simulink model "amrNavigation"  (R2025b)
settings: Solver=FixedStepDiscrete  StartTime=0.0  StopTime=119.95  FixedStep=0.050000000000000003  RelTol=1e-3
InitFcn:
  | amrModelInit
StopFcn:
  | amrModelStop
model workspace (MAT data in the model file):
  amrBuiltConstants.robot.radius = 0.22
  amrBuiltConstants.robot.wheelRadius = 0.05
  amrBuiltConstants.robot.wheelBase = 0.32
  amrBuiltConstants.robot.vMax = 0.65
  amrBuiltConstants.robot.vMin = -0.2
  amrBuiltConstants.robot.wMax = 1.4
  amrBuiltConstants.robot.aMax = 0.6
  amrBuiltConstants.robot.alphaMax = 2
  amrBuiltConstants.robot.motorTau = 0.06
  amrBuiltConstants.robot.wheelSpeedMax = 25
  amrBuiltConstants.robot.idealWheels = 0
  amrBuiltConstants.robot.integrator = 'euler'
  amrBuiltConstants.wheelPID.Kp = 0.5
  amrBuiltConstants.wheelPID.Ki = 3
  amrBuiltConstants.wheelPID.Kd = 0
  amrBuiltConstants.wheelPID.iMax = 10
  amrBuiltConstants.dt = 0.05
undefined symbols (not defined in the file or in its folder): amrStartPose
libraries: simulink x1
settings Model: Creator=kichuiyer  LastModifiedBy=kichuiyer
settings DataIOCC: SaveOutput=off  SignalLogging=off  SaveTime=off

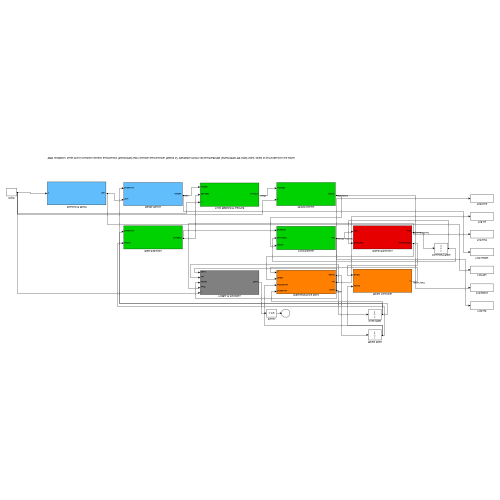
[thumbnail: Simulink's stored preview of the top-level diagram]
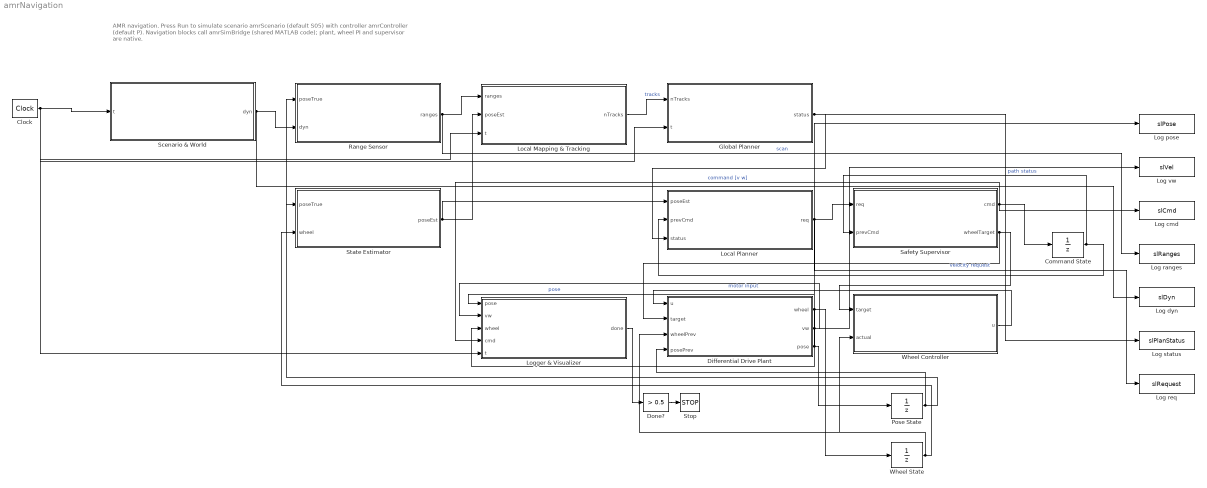
== system amrNavigation ==
  note: AMR navigation. Press Run to simulate scenario amrScenario (default S05) with controller amrController (default P). Navigation blocks call amrSimBridge (shared MATLAB code); plant, wheel PI and supervisor are native.
  Clock : DigitalClock  SampleTime=0.050000000000000003
  Command State : UnitDelay  InitialCondition=[0 0]  SampleTime=0.050000000000000003  HasFrameUpgradeWarning=on
  Differential Drive Plant : Subsystem
  Done? : simulink/Logic and Bit Operations/Compare To Constant  relop=>  const=0.5  OutDataTypeStr=boolean
  Global Planner : Subsystem
  Local Mapping & Tracking : Subsystem
  Local Planner : Subsystem
  Log cmd : ToWorkspace  VariableName=slCmd  SampleTime=-1
  Log dyn : ToWorkspace  VariableName=slDyn  SampleTime=-1
  Log pose : ToWorkspace  VariableName=slPose  SampleTime=-1
  Log ranges : ToWorkspace  VariableName=slRanges  SampleTime=-1
  Log req : ToWorkspace  VariableName=slRequest  SampleTime=-1
  Log status : ToWorkspace  VariableName=slPlanStatus  SampleTime=-1
  Log vw : ToWorkspace  VariableName=slVel  SampleTime=-1
  Logger & Visualizer : Subsystem
  Pose State : UnitDelay  InitialCondition=amrStartPose  SampleTime=0.050000000000000003  HasFrameUpgradeWarning=on
  Range Sensor : Subsystem
  Safety Supervisor : Subsystem
  Scenario & World : Subsystem
  State Estimator : Subsystem
  Stop : Stop
  Wheel Controller : Subsystem
  Wheel State : UnitDelay  InitialCondition=[0 0]  SampleTime=0.050000000000000003  HasFrameUpgradeWarning=on
  wires:
  Clock/1 -> Scenario & World/1(t), Local Mapping & Tracking/3(t), Global Planner/2(t), Logger & Visualizer/5(t)
  Scenario & World/1(dyn) -> Range Sensor/2(dyn), Log dyn/1
  Pose State/1 -> Range Sensor/1(poseTrue), State Estimator/1(poseTrue), Differential Drive Plant/4(posePrev)
  Wheel State/1 -> State Estimator/2(wheel), Wheel Controller/2(actual), Differential Drive Plant/3(wheelPrev)
  Range Sensor/1(ranges) -> Local Mapping & Tracking/1(ranges), Log ranges/1  "scan"
  State Estimator/1(poseEst) -> Local Mapping & Tracking/2(poseEst), Local Planner/1(poseEst)
  Local Mapping & Tracking/1(nTracks) -> Global Planner/1(nTracks)  "tracks"
  Command State/1 -> Local Planner/2(prevCmd), Safety Supervisor/2(prevCmd)
  Global Planner/1(status) -> Local Planner/3(status), Log status/1  "path status"
  Local Planner/1(req) -> Safety Supervisor/1(req), Log req/1  "velocity request"
  Safety Supervisor/1(cmd) -> Command State/1, Logger & Visualizer/4(cmd), Log cmd/1  "command [v w]"
  Safety Supervisor/2(wheelTarget) -> Wheel Controller/1(target), Differential Drive Plant/2(target)
  Wheel Controller/1(u) -> Differential Drive Plant/1(u)  "motor input"
  Differential Drive Plant/1(wheel) -> Wheel State/1, Logger & Visualizer/3(wheel)
  Differential Drive Plant/3(pose) -> Pose State/1, Logger & Visualizer/1(pose), Log pose/1  "pose"
  Differential Drive Plant/2(vw) -> Logger & Visualizer/2(vw), Log vw/1
  Logger & Visualizer/1(done) -> Done?/1
  Done?/1 -> Stop/1

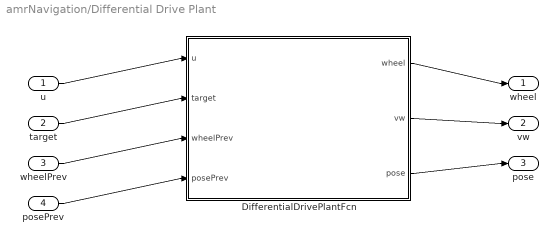
== system amrNavigation/Differential Drive Plant ==
  u : Inport
  target : Inport  Port=2
  wheelPrev : Inport  Port=3
  posePrev : Inport  Port=4
  DifferentialDrivePlantFcn : MATLAB Function  TreatAsAtomicUnit=on
  wheel : Outport
  vw : Outport  Port=2
  pose : Outport  Port=3
  wires:
  u/1 -> DifferentialDrivePlantFcn/1(u)
  target/1 -> DifferentialDrivePlantFcn/2(target)
  wheelPrev/1 -> DifferentialDrivePlantFcn/3(wheelPrev)
  posePrev/1 -> DifferentialDrivePlantFcn/4(posePrev)
  DifferentialDrivePlantFcn/1(wheel) -> wheel/1
  DifferentialDrivePlantFcn/2(vw) -> vw/1
  DifferentialDrivePlantFcn/3(pose) -> pose/1

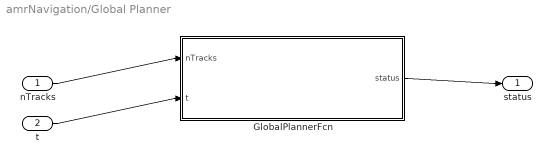
== system amrNavigation/Global Planner ==
  nTracks : Inport
  t : Inport  Port=2
  GlobalPlannerFcn : MATLAB Function  TreatAsAtomicUnit=on
  status : Outport
  wires:
  nTracks/1 -> GlobalPlannerFcn/1(nTracks)
  t/1 -> GlobalPlannerFcn/2(t)
  GlobalPlannerFcn/1(status) -> status/1

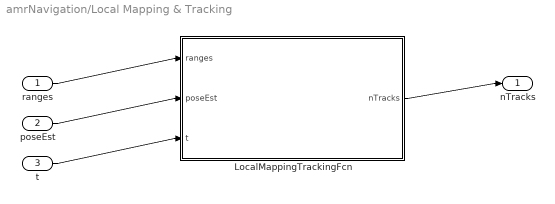
== system amrNavigation/Local Mapping & Tracking ==
  ranges : Inport
  poseEst : Inport  Port=2
  t : Inport  Port=3
  LocalMappingTrackingFcn : MATLAB Function  TreatAsAtomicUnit=on
  nTracks : Outport
  wires:
  ranges/1 -> LocalMappingTrackingFcn/1(ranges)
  poseEst/1 -> LocalMappingTrackingFcn/2(poseEst)
  t/1 -> LocalMappingTrackingFcn/3(t)
  LocalMappingTrackingFcn/1(nTracks) -> nTracks/1

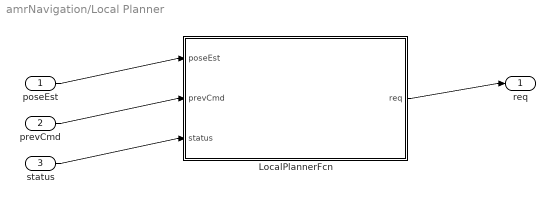
== system amrNavigation/Local Planner ==
  poseEst : Inport
  prevCmd : Inport  Port=2
  status : Inport  Port=3
  LocalPlannerFcn : MATLAB Function  TreatAsAtomicUnit=on
  req : Outport
  wires:
  poseEst/1 -> LocalPlannerFcn/1(poseEst)
  prevCmd/1 -> LocalPlannerFcn/2(prevCmd)
  status/1 -> LocalPlannerFcn/3(status)
  LocalPlannerFcn/1(req) -> req/1

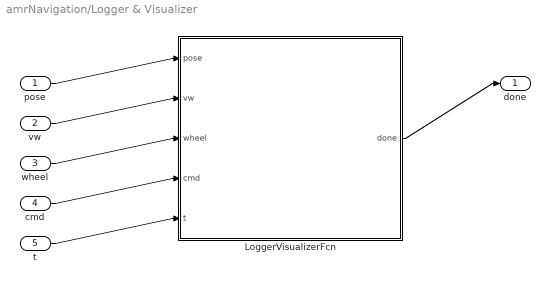
== system amrNavigation/Logger & Visualizer ==
  pose : Inport
  vw : Inport  Port=2
  wheel : Inport  Port=3
  cmd : Inport  Port=4
  t : Inport  Port=5
  LoggerVisualizerFcn : MATLAB Function  TreatAsAtomicUnit=on
  done : Outport
  wires:
  pose/1 -> LoggerVisualizerFcn/1(pose)
  vw/1 -> LoggerVisualizerFcn/2(vw)
  wheel/1 -> LoggerVisualizerFcn/3(wheel)
  cmd/1 -> LoggerVisualizerFcn/4(cmd)
  t/1 -> LoggerVisualizerFcn/5(t)
  LoggerVisualizerFcn/1(done) -> done/1

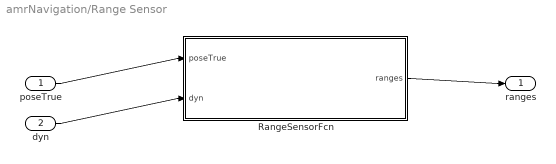
== system amrNavigation/Range Sensor ==
  poseTrue : Inport
  dyn : Inport  Port=2
  RangeSensorFcn : MATLAB Function  TreatAsAtomicUnit=on
  ranges : Outport
  wires:
  poseTrue/1 -> RangeSensorFcn/1(poseTrue)
  dyn/1 -> RangeSensorFcn/2(dyn)
  RangeSensorFcn/1(ranges) -> ranges/1

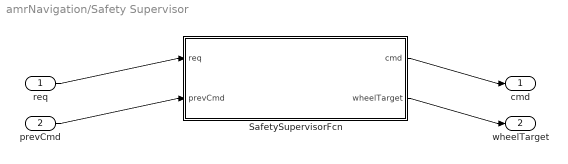
== system amrNavigation/Safety Supervisor ==
  req : Inport
  prevCmd : Inport  Port=2
  SafetySupervisorFcn : MATLAB Function  TreatAsAtomicUnit=on
  cmd : Outport
  wheelTarget : Outport  Port=2
  wires:
  req/1 -> SafetySupervisorFcn/1(req)
  prevCmd/1 -> SafetySupervisorFcn/2(prevCmd)
  SafetySupervisorFcn/1(cmd) -> cmd/1
  SafetySupervisorFcn/2(wheelTarget) -> wheelTarget/1

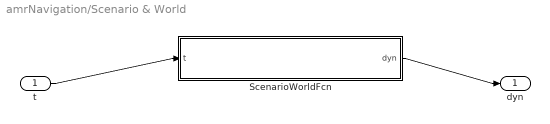
== system amrNavigation/Scenario & World ==
  t : Inport
  ScenarioWorldFcn : MATLAB Function  TreatAsAtomicUnit=on
  dyn : Outport
  wires:
  t/1 -> ScenarioWorldFcn/1(t)
  ScenarioWorldFcn/1(dyn) -> dyn/1

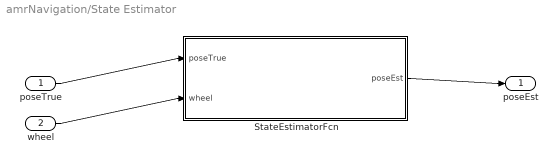
== system amrNavigation/State Estimator ==
  poseTrue : Inport
  wheel : Inport  Port=2
  StateEstimatorFcn : MATLAB Function  TreatAsAtomicUnit=on
  poseEst : Outport
  wires:
  poseTrue/1 -> StateEstimatorFcn/1(poseTrue)
  wheel/1 -> StateEstimatorFcn/2(wheel)
  StateEstimatorFcn/1(poseEst) -> poseEst/1

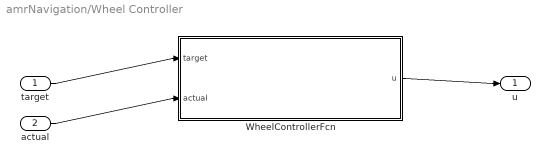
== system amrNavigation/Wheel Controller ==
  target : Inport
  actual : Inport  Port=2
  WheelControllerFcn : MATLAB Function  TreatAsAtomicUnit=on
  u : Outport
  wires:
  target/1 -> WheelControllerFcn/1(target)
  actual/1 -> WheelControllerFcn/2(actual)
  WheelControllerFcn/1(u) -> u/1

== matlab function amrNavigation/Range Sensor/RangeSensorFcn ==
  data: poseTrue input; ranges output; dyn input
function ranges = fcn(poseTrue, dyn)
%#codegen
% Range Sensor: ray-cast LiDAR from the TRUE pose (-1 = no return)
coder.extrinsic('amrSimBridge');
ranges = zeros(1, 181);
ranges = amrSimBridge('sense', reshape(poseTrue, 1, 3));
end

== matlab function amrNavigation/Scenario & World/ScenarioWorldFcn ==
  data: t input; dyn output
function dyn = fcn(t)
%#codegen
% Scenario & World: advance scripted obstacles and hidden blockers (ground truth)
coder.extrinsic('amrSimBridge');
dyn = zeros(1, 18);
dyn = amrSimBridge('world', t);
end

== matlab function amrNavigation/State Estimator/StateEstimatorFcn ==
  data: poseTrue input; poseEst output; wheel input
function poseEst = fcn(poseTrue, wheel)
%#codegen
% State Estimator: exact pose (cfg.odom.useTruePose = true baseline).
% Replace with odometry / localisation to study estimation error.
poseEst = reshape(poseTrue, 1, 3);
end

== matlab function amrNavigation/Local Mapping & Tracking/LocalMappingTrackingFcn ==
  data: ranges input; nTracks output; poseEst input; t input
function nTracks = fcn(ranges, poseEst, t)
%#codegen
% Local Mapping & Tracking: clustering, alpha-beta tracks, observed-obstacle grid
coder.extrinsic('amrSimBridge');
nTracks = zeros(1, 2);
nTracks = amrSimBridge('perceive', reshape(poseEst, 1, 3), t);
end

== matlab function amrNavigation/Global Planner/GlobalPlannerFcn ==
  data: nTracks input; status output; t input
function status = fcn(nTracks, t)
%#codegen
% Global Planner: blockage detection, debounced A* replanning
% status = [nWaypoints blocked replans]
coder.extrinsic('amrSimBridge');
status = zeros(1, 3);
status = amrSimBridge('replan', t);
end

== matlab function amrNavigation/Local Planner/LocalPlannerFcn ==
  data: poseEst input; req output; prevCmd input; status input
function req = fcn(poseEst, prevCmd, status)
%#codegen
% Local Planner: look-ahead tracking + DWA-style velocity sampling
% req = [vRequest wRequest mode]  (mode 0 normal, 1 evasive, 2 stop)
coder.extrinsic('amrSimBridge');
req = zeros(1, 3);
req = amrSimBridge('command', reshape(poseEst, 1, 3), reshape(prevCmd, 1, 2));
end

== matlab function amrNavigation/Safety Supervisor/SafetySupervisorFcn ==
  data: req input; cmd output; prevCmd input; wheelTarget output
function [cmd, wheelTarget] = fcn(req, prevCmd)
%#codegen
% Safety Supervisor: speed and acceleration limits (limitCommand), then
% inverse kinematics to wheel speed targets.
dt = 0.050000000000000003; vMin = -0.20000000000000001; vMax = 0.65000000000000002; wMax = 1.3999999999999999; aMax = 0.59999999999999998; alphaMax = 2;
r = 0.050000000000000003; b = 0.32000000000000001;
v = min(max(req(1), vMin), vMax);
w = min(max(req(2), -wMax), wMax);
v = min(max(v, prevCmd(1) - aMax * dt), prevCmd(1) + aMax * dt);
w = min(max(w, prevCmd(2) - alphaMax * dt), prevCmd(2) + alphaMax * dt);
cmd = [v w];
wheelTarget = [(cmd(1) + cmd(2) * b / 2) / r, (cmd(1) - cmd(2) * b / 2) / r];
end

== matlab function amrNavigation/Wheel Controller/WheelControllerFcn ==
  data: target input; u output; actual input
function u = fcn(target, actual)
%#codegen
% Wheel Controller: PI(D) with feedforward and conditional-integration anti-windup
persistent integ prevErr
if isempty(integ), integ = [0 0]; prevErr = [0 0]; end
dt = 0.050000000000000003; Kp = 0.5; Ki = 3; Kd = 0; iMax = 10; uMax = 25;
target = reshape(target, 1, 2); actual = reshape(actual, 1, 2);
e = target - actual;
integCand = integ + e * dt;
integCand = min(max(integCand, -iMax / max(Ki, eps)), iMax / max(Ki, eps));
d = (e - prevErr) / dt;
uCand = target + Kp * e + Ki * integCand + Kd * d;
sat = abs(uCand) > uMax;
newInteg = integCand;
for i = 1:2
    if sat(i), newInteg(i) = integ(i); end
end
u = target + Kp * e + Ki * newInteg + Kd * d;
u = min(max(u, -uMax), uMax);
integ = newInteg; prevErr = e;
end

== matlab function amrNavigation/Differential Drive Plant/DifferentialDrivePlantFcn ==
  data: u input; wheel output; target input; wheelPrev input; posePrev input; vw output; pose output
function [wheel, vw, pose] = fcn(u, target, wheelPrev, posePrev)
%#codegen
% Differential Drive Plant: first-order wheel motors (exact ZOH),
% v = r/2 (wR + wL), w = r/b (wR - wL), pose integration, yaw wrap.
dt = 0.050000000000000003; tau = 0.059999999999999998; r = 0.050000000000000003; b = 0.32000000000000001;
u = reshape(u, 1, 2); target = reshape(target, 1, 2); wheelPrev = reshape(wheelPrev, 1, 2);
a = 1 - exp(-dt / tau);
wheel = wheelPrev + a * (u - wheelPrev);
wheel = min(max(wheel, -25), 25);
v = r / 2 * (wheel(1) + wheel(2));
w = r / b * (wheel(1) - wheel(2));
p = reshape(posePrev, 1, 3);
pose = [p(1) + v * cos(p(3)) * dt, p(2) + v * sin(p(3)) * dt, p(3) + w * dt];
pose(3) = mod(pose(3) + pi, 2*pi) - pi;
vw = [v w];
end

== matlab function amrNavigation/Logger & Visualizer/LoggerVisualizerFcn ==
  data: pose input; done output; vw input; wheel input; cmd input; t input
function done = fcn(pose, vw, wheel, cmd, t)
%#codegen
% Logger: ground-truth collision / goal / failure checks and run log
coder.extrinsic('amrSimBridge');
done = 0;
done = amrSimBridge('post', reshape(pose, 1, 3), reshape(vw, 1, 2), reshape(wheel, 1, 2), reshape(cmd, 1, 2), t);
end
